simulink subsystem "joystick"  (R2026a)
settings: Solver=VariableStepAuto
undefined symbols (not defined in the file): DiscIntNeverNeededParam, FF_maneuvers, I, P, RSFF_maneuvers, S, T
libraries: slpidlib x2, simulink x1
settings Model: Creator=rubystanton  LastModifiedBy=kjhaydon

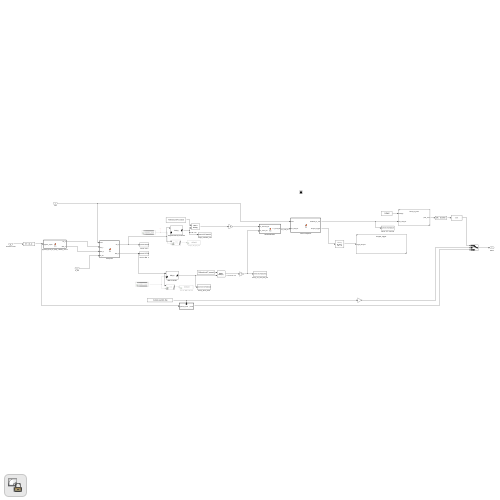
[thumbnail: Simulink's stored preview of the top-level diagram]
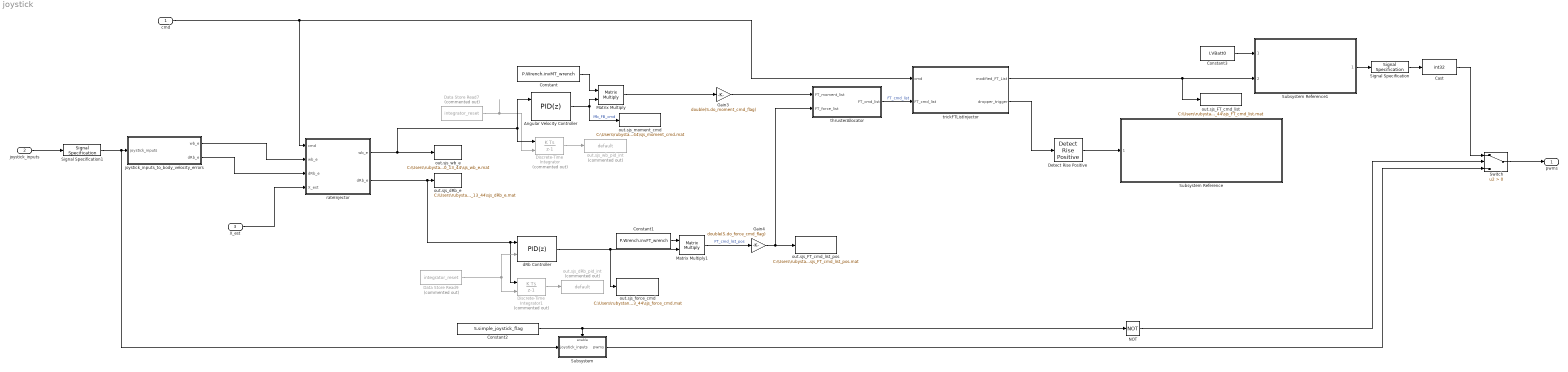
== system joystick ==
  cmd : Inport
  joystick_inputs : Inport  Port=2
  X_est : Inport  Port=3
  Angular Velocity Controller : slpidlib/PID Controller  Controller=PID  Form=Parallel  TimeDomain=Discrete-time  UseExternalTs=off  SampleTime=-1  IntegratorMethod=Forward Euler  FilterMethod=Forward Euler  ControllerParametersSource=internal  P=T.wb_PID.Kp  I=T.wb_PID.Ki  UseKiTs=off  D=T.wb_PID.Kd  UseExternalDerivativeSource=off  N=T.wb_PID.N  UseFilter=on  TunerSelectOption=Transfer Function Based (PID Tuner App)  InitialConditionSource=internal  InitialConditionForIntegrator=0  InitialConditionForFilter=0  DifferentiatorICPrevScaledInput=0  ExternalReset=rising  TrackingMode=off  Kt=1  LimitOutput=on  SatLimitsSource=internal  UpperSaturationLimit=T.wb_PID.output_sat  LowerSaturationLimit=-T.wb_PID.output_sat  LinearizeAsGain=on  AntiWindupMode=clamping  Kb=1  LimitIntegrator=on  UpperIntegratorSaturationLimit=T.wb_PID.int_sat  LowerIntegratorSaturationLimit=-T.wb_PID.int_sat  POutMin=[]  POutMax=[]  IOutMin=[]  IOutMax=[]  DOutMin=[]  DOutMax=[]  NOutMin=[]  NOutMax=[]  SumOutMin=[]  SumOutMax=[]  SaturationOutMin=[]  SaturationOutMax=[]  PParamMin=[]  PParamMax=[]  IParamMin=[]  IParamMax=[]  DParamMin=[]  DParamMax=[]  NParamMin=[]  NParamMax=[]  KbParamMin=[]  KbParamMax=[]  KtParamMin=[]  KtParamMax=[]  KbOutMin=[]  KbOutMax=[]  KtOutMin=[]  KtOutMax=[]  IntegratorOutMin=[]  IntegratorOutMax=[]  FilterOutMin=[]  FilterOutMax=[]  SumI1OutMin=[]  SumI1OutMax=[]  SumI2OutMin=[]  SumI2OutMax=[]  SumI3OutMin=[]  SumI3OutMax=[]  SumI4OutMin=[]  SumI4OutMax=[]  SumDOutMin=[]  SumDOutMax=[]  DifferentiatorOutMin=[]  DifferentiatorOutMax=[]  FilterDiffOutCoefMin=[]  FilterDiffOutCoefMax=[]  ReciprocalOutMin=[]  ReciprocalOutMax=[]  SumDenOutMin=[]  SumDenOutMax=[]  SumNumOutMin=[]  SumNumOutMax=[]  DivideOutMin=[]  DivideOutMax=[]  UdiffTsProdOutMin=[]  UdiffTsProdOutMax=[]  NTsProdOutMin=[]  NTsProdOutMax=[]  UintegralTsProdOutMin=[]  UintegralTsProdOutMax=[]  UngainTsProdOutMin=[]  UngainTsProdOutMax=[]  ClampingZeroOutDataTypeStr=Inherit: Inherit via back propagation  ClampingZeroOutMin=[]  ClampingZeroOutMax=[]  FilterDenConstantOutDataTypeStr=Inherit: Inherit via back propagation  FilterDenConstantOutMin=[]  FilterDenConstantOutMax=[]  PCopyOutDataTypeStr=Inherit: Inherit via back propagation  PCopyOutMin=[]  PCopyOutMax=[]  NCopyOutDataTypeStr=Inherit: Inherit via back propagation  NCopyOutMin=[]  NCopyOutMax=[]  IntegratorContinuousStateAttributes=''  IntegratorStateMustResolveToSignalObject=off  IntegratorRTWStateStorageClass=Auto  FilterContinuousStateAttributes=''  FilterStateMustResolveToSignalObject=off  FilterRTWStateStorageClass=Auto  ParallelPVariant=InternalParameters  IdealPVariant=Disabled  IVariant=InternalParameters  DVariant=InternalParameters  IntegratorVariant=Discrete  SatVariant=Enabled  AWVariant=DiscClampingParallel  PCopyVariant=Disabled  TRVariant=Disabled  FdbkBlocksVariant=Forward  IdealPFdbkVariant=Disabled  SatFdbkVariant=Disabled  DerivativeFilterVariant=ForwardEulerFilter  NVariant=InternalParameters  NCopyVariant=Disabled  FilterICVariant=InternalICsFilter  IntegratorICVariant=InternalICs  ExternalResetVariant=ExternalReset  TRSumVariant=Passthrough  SumFdbkVariant=Disabled  SumVariant=Sum_PID  TsampFilterVariant=InternalTs  TsampNgainVariant=Passthrough  TsampIntegralVariant=Disabled_SignalSpec  ExternalSaturationOutDataTypeStr=Inherit: Same as second input  DerivativeSourceVariant=ErrorSignal  PreIntVariant=InternalPreInt
  Cast : DataTypeConversion  OutDataTypeStr=int32  SaturateOnIntegerOverflow=off  RndMeth=Floor
  Constant : Constant  Value=P.Wrench.invMT_wrench
  Constant1 : Constant  Value=P.Wrench.invFT_wrench
  Constant2 : Constant  Value=S.simple_joystick_flag
  Constant3 : Constant  Value=I.VBatt0
  Data Store Read7 : DataStoreRead  Commented=on  DataStoreName=integrator_reset  IndexOptions=Index vector (dialog)  Indices=1  OutputSizes=1
  Data Store Read9 : DataStoreRead  Commented=on  DataStoreName=integrator_reset  IndexOptions=Index vector (dialog)  Indices=1  OutputSizes=1
  Detect Rise Positive : simulink/Logic and Bit Operations/Detect Rise Positive  vinit=0  OutDataTypeStr=boolean
  Discrete-Time Integrator : DiscreteIntegrator  Commented=on  gainval=T.wb_PID.Ki  ExternalReset=rising  InitialCondition=[0;0;0]  SampleTime=S.dt_control  LimitOutput=on  UpperSaturationLimit=T.wb_PID.int_sat  LowerSaturationLimit=-T.wb_PID.int_sat  ICPrevOutput=DiscIntNeverNeededParam  ICPrevScaledInput=DiscIntNeverNeededParam
  Discrete-Time Integrator1 : DiscreteIntegrator  Commented=on  gainval=T.dRb_PID.Ki  ExternalReset=rising  InitialCondition=[0;0;0]  SampleTime=S.dt_control  LimitOutput=on  UpperSaturationLimit=T.dRb_PID.int_sat  LowerSaturationLimit=-T.dRb_PID.int_sat  ICPrevOutput=DiscIntNeverNeededParam  ICPrevScaledInput=DiscIntNeverNeededParam
  Gain3 : Gain  Gain=double(S.do_moment_cmd_flag)
  Gain4 : Gain  Gain=double(S.do_force_cmd_flag)
  Matrix Multiply : Product  Multiplication=Matrix(*)
  Matrix Multiply1 : Product  Multiplication=Matrix(*)
  NOT : Logic  Operator=NOT  IconShape=distinctive  AllPortsSameDT=off  OutDataTypeStr=boolean
  Signal Specification : SignalSpecification  OutDataTypeStr=double
  Signal Specification1 : SignalSpecification  Dimensions=[6,1]
  Subsystem : Subsystem
  Subsystem Reference : Subsystem  ReferencedSubsystem=dropper_trigger
  Subsystem Reference1 : Subsystem  ReferencedSubsystem=force_to_pwm
  Switch : Switch  Criteria=u2 > Threshold  SaturateOnIntegerOverflow=off  InputSameDT=off
  dRb Controller : slpidlib/PID Controller  Controller=PID  Form=Parallel  TimeDomain=Discrete-time  UseExternalTs=off  SampleTime=-1  IntegratorMethod=Forward Euler  FilterMethod=Forward Euler  ControllerParametersSource=internal  P=T.dRb_PID.Kp  I=T.dRb_PID.Ki  UseKiTs=off  D=T.dRb_PID.Kd  UseExternalDerivativeSource=off  N=T.dRb_PID.N  UseFilter=on  TunerSelectOption=Transfer Function Based (PID Tuner App)  InitialConditionSource=internal  InitialConditionForIntegrator=0  InitialConditionForFilter=0  DifferentiatorICPrevScaledInput=0  ExternalReset=rising  TrackingMode=off  Kt=1  LimitOutput=on  SatLimitsSource=internal  UpperSaturationLimit=T.dRb_PID.output_sat  LowerSaturationLimit=-T.dRb_PID.output_sat  LinearizeAsGain=on  AntiWindupMode=clamping  Kb=1  LimitIntegrator=on  UpperIntegratorSaturationLimit=T.dRb_PID.int_sat  LowerIntegratorSaturationLimit=-T.dRb_PID.int_sat  POutMin=[]  POutMax=[]  IOutMin=[]  IOutMax=[]  DOutMin=[]  DOutMax=[]  NOutMin=[]  NOutMax=[]  SumOutMin=[]  SumOutMax=[]  SaturationOutMin=[]  SaturationOutMax=[]  PParamMin=[]  PParamMax=[]  IParamMin=[]  IParamMax=[]  DParamMin=[]  DParamMax=[]  NParamMin=[]  NParamMax=[]  KbParamMin=[]  KbParamMax=[]  KtParamMin=[]  KtParamMax=[]  KbOutMin=[]  KbOutMax=[]  KtOutMin=[]  KtOutMax=[]  IntegratorOutMin=[]  IntegratorOutMax=[]  FilterOutMin=[]  FilterOutMax=[]  SumI1OutMin=[]  SumI1OutMax=[]  SumI2OutMin=[]  SumI2OutMax=[]  SumI3OutMin=[]  SumI3OutMax=[]  SumI4OutMin=[]  SumI4OutMax=[]  SumDOutMin=[]  SumDOutMax=[]  DifferentiatorOutMin=[]  DifferentiatorOutMax=[]  FilterDiffOutCoefMin=[]  FilterDiffOutCoefMax=[]  ReciprocalOutMin=[]  ReciprocalOutMax=[]  SumDenOutMin=[]  SumDenOutMax=[]  SumNumOutMin=[]  SumNumOutMax=[]  DivideOutMin=[]  DivideOutMax=[]  UdiffTsProdOutMin=[]  UdiffTsProdOutMax=[]  NTsProdOutMin=[]  NTsProdOutMax=[]  UintegralTsProdOutMin=[]  UintegralTsProdOutMax=[]  UngainTsProdOutMin=[]  UngainTsProdOutMax=[]  ClampingZeroOutDataTypeStr=Inherit: Inherit via back propagation  ClampingZeroOutMin=[]  ClampingZeroOutMax=[]  FilterDenConstantOutDataTypeStr=Inherit: Inherit via back propagation  FilterDenConstantOutMin=[]  FilterDenConstantOutMax=[]  PCopyOutDataTypeStr=Inherit: Inherit via back propagation  PCopyOutMin=[]  PCopyOutMax=[]  NCopyOutDataTypeStr=Inherit: Inherit via back propagation  NCopyOutMin=[]  NCopyOutMax=[]  IntegratorContinuousStateAttributes=''  IntegratorStateMustResolveToSignalObject=off  IntegratorRTWStateStorageClass=Auto  FilterContinuousStateAttributes=''  FilterStateMustResolveToSignalObject=off  FilterRTWStateStorageClass=Auto  ParallelPVariant=InternalParameters  IdealPVariant=Disabled  IVariant=InternalParameters  DVariant=InternalParameters  IntegratorVariant=Discrete  SatVariant=Enabled  AWVariant=DiscClampingParallel  PCopyVariant=Disabled  TRVariant=Disabled  FdbkBlocksVariant=Forward  IdealPFdbkVariant=Disabled  SatFdbkVariant=Disabled  DerivativeFilterVariant=ForwardEulerFilter  NVariant=InternalParameters  NCopyVariant=Disabled  FilterICVariant=InternalICsFilter  IntegratorICVariant=InternalICs  ExternalResetVariant=ExternalReset  TRSumVariant=Passthrough  SumFdbkVariant=Disabled  SumVariant=Sum_PID  TsampFilterVariant=InternalTs  TsampNgainVariant=Passthrough  TsampIntegralVariant=Disabled_SignalSpec  ExternalSaturationOutDataTypeStr=Inherit: Same as second input  DerivativeSourceVariant=ErrorSignal  PreIntVariant=InternalPreInt
  joystick_inputs_to_body_velocity_errors : MATLAB Function  TreatAsAtomicUnit=on
  out.sjs_FT_cmd_list : ToFile  Filename=C:\Users\rubystanton\Documents\GitHub\controls-2027\data\2026_10_27_20_13_44\sjs_FT_cmd_list.mat  MatrixName=sjs_FT_cmd_list  SaveFormat=Timeseries  SampleTime=S.dt_data
  out.sjs_FT_cmd_list_pos : ToFile  Filename=C:\Users\rubystanton\Documents\GitHub\controls-2027\data\2026_10_27_20_13_44\sjs_FT_cmd_list_pos.mat  MatrixName=sjs_FT_cmd_list_pos  SaveFormat=Timeseries
  out.sjs_dRb_e : ToFile  Filename=C:\Users\rubystanton\Documents\GitHub\controls-2027\data\2026_10_27_20_13_44\sjs_dRb_e.mat  MatrixName=sjs_dRb_e  SaveFormat=Timeseries  SampleTime=S.dt_data
  out.sjs_dRb_pid_int : ToFile  Commented=on  Filename=default  MatrixName=sjs_dRb_pid_int  SaveFormat=Timeseries  SampleTime=S.dt_data
  out.sjs_force_cmd : ToFile  Filename=C:\Users\rubystanton\Documents\GitHub\controls-2027\data\2026_10_27_20_13_44\sjs_force_cmd.mat  MatrixName=sjs_force_cmd  SaveFormat=Timeseries  SampleTime=S.dt_data
  out.sjs_moment_cmd : ToFile  Filename=C:\Users\rubystanton\Documents\GitHub\controls-2027\data\2026_10_27_20_13_44\sjs_moment_cmd.mat  MatrixName=sjs_moment_cmd  SaveFormat=Timeseries  SampleTime=S.dt_data
  out.sjs_wb_e : ToFile  Filename=C:\Users\rubystanton\Documents\GitHub\controls-2027\data\2026_10_27_20_13_44\sjs_wb_e.mat  MatrixName=sjs_wb_e  SaveFormat=Timeseries  SampleTime=S.dt_data
  out.sjs_wb_pid_int : ToFile  Commented=on  Filename=default  MatrixName=sjs_wb_pid_int  SaveFormat=Timeseries  SampleTime=S.dt_data
  rateInjector : MATLAB Function  TreatAsAtomicUnit=on
  thrusterAllocator : MATLAB Function  TreatAsAtomicUnit=on
  trickFTListInjector : MATLAB Function  TreatAsAtomicUnit=on
  pwms : Outport
  wires:
  trickFTListInjector/2(dropper_trigger) -> Detect Rise Positive/1
  Subsystem/1(pwms) -> Switch/3
  NOT/1 -> Switch/2
  Signal Specification/1 -> Cast/1
  Matrix Multiply/1 -> Gain3/1
  Signal Specification1/1 -> Subsystem/1(joystick_inputs), joystick_inputs_to_body_velocity_errors/1(joystick_inputs)
  Detect Rise Positive/1 -> Subsystem Reference/1
  thrusterAllocator/1(FT_cmd_list) -> trickFTListInjector/2(FT_cmd_list)  "FT_cmd_list"
  Subsystem Reference1/1 -> Signal Specification/1
  Discrete-Time Integrator/1 -> out.sjs_wb_pid_int/1
  Discrete-Time Integrator1/1 -> out.sjs_dRb_pid_int/1
  Switch/1 -> pwms/1
  cmd/1 -> rateInjector/1(cmd), trickFTListInjector/1(cmd)
  Data Store Read7/1 -> Discrete-Time Integrator/2
  X_est/1 -> rateInjector/4(X_est)
  Constant/1 -> Matrix Multiply/1
  Constant2/1 -> NOT/1, Subsystem/Enable
  rateInjector/2(dRb_e) -> out.sjs_dRb_e/1, Discrete-Time Integrator1/1, dRb Controller/1
  dRb Controller/1 -> Matrix Multiply1/2, out.sjs_force_cmd/1
  Angular Velocity Controller/1 -> Matrix Multiply/2, out.sjs_moment_cmd/1  "Mb_FB_cmd"
  Constant3/1 -> Subsystem Reference1/1
  Data Store Read9/1 -> dRb Controller/2, Discrete-Time Integrator1/2
  joystick_inputs_to_body_velocity_errors/1(wb_e) -> rateInjector/2("wb_e ")
  joystick_inputs/1 -> Signal Specification1/1
  Constant1/1 -> Matrix Multiply1/1
  Gain3/1 -> thrusterAllocator/1(FT_moment_list)
  rateInjector/1(wb_e) -> out.sjs_wb_e/1, Discrete-Time Integrator/1, Angular Velocity Controller/1
  joystick_inputs_to_body_velocity_errors/2(dRb_e) -> rateInjector/3("dRb_e ")
  Cast/1 -> Switch/1
  Matrix Multiply1/1 -> Gain4/1  "FT_cmd_list_pos"
  Gain4/1 -> out.sjs_FT_cmd_list_pos/1, thrusterAllocator/2(FT_force_list)
  trickFTListInjector/1(modified_FT_List) -> out.sjs_FT_cmd_list/1, Subsystem Reference1/2

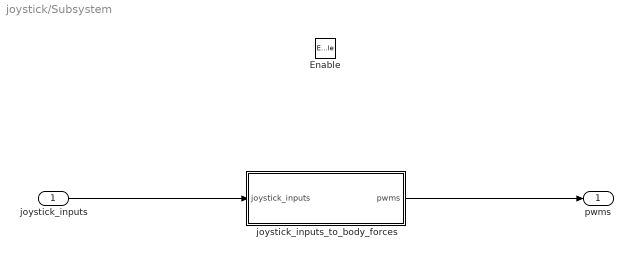
== system joystick/Subsystem ==
  joystick_inputs : Inport
  Enable : EnablePort
  joystick_inputs_to_body_forces : MATLAB Function  TreatAsAtomicUnit=on
  pwms : Outport
  wires:
  joystick_inputs_to_body_forces/1(pwms) -> pwms/1
  joystick_inputs/1 -> joystick_inputs_to_body_forces/1(joystick_inputs)

== matlab function joystick/Subsystem/joystick_inputs_to_body_forces ==
  data: pwms output; joystick_inputs input
%{
Function ported from SimulinkPlant Kory-Work-Branch Mission_Manager_HIL.slx.

Written by Alex Zamora.
%}

function pwms = fcn(joystick_inputs)

%Create the mapping here for PWM values.
%Recall that PWM 1-8 correspond to thruster postions which follow,

%pwm of each thruster on the robot
%In left to right:
%f = front / r = rear
%l = left  / r = right
%t = top   / b = bottom
%PWM(1)=pwm_flt
%PWM(2)=pwm_frt
%PWM(3)=pwm_rlt
%PWM(4)=pwm_rrt
%PWM(5)=pwm_flb
%PWM(6)=pwm_frb
%PWM(7)=pwm_rlb
%PWM(8)=pwm_rrb
  
x_joy = joystick_inputs(1);
y_joy = joystick_inputs(2);
rise = joystick_inputs(3);
sink = joystick_inputs(4);
yaw = joystick_inputs(5);
pitch = joystick_inputs(6);


scale = 300;
stop_set = 1500;
max_pwm = 1500+scale;
min_pwm = 1500-scale;

%x_body and y_body mapping
x = y_joy;
y = x_joy;

pwms_vert = stop_set*ones(1,4); %Thrusters 0,1,2,3
pwms_horiz = stop_set*ones(1,4); %Thrusters 4,5,6,7
inversion_mask = [1, -1, 1, -1];

% Rise/Sink
for i = 1:4
    pwms_vert(i) = pwms_vert(i) + (scale*rise - scale*sink) * inversion_mask(i);
end

%Pitch
pwms_vert(1) = pwms_vert(1) - (scale*pitch*inversion_mask(1));
pwms_vert(2) = pwms_vert(2) - (scale*pitch*inversion_mask(2));
pwms_vert(3) = pwms_vert(3) + (scale*pitch*inversion_mask(3));
pwms_vert(4) = pwms_vert(4) + (scale*pitch*inversion_mask(4));

% Forwards:
pwms_horiz(1) = pwms_horiz(1) + scale*x;
pwms_horiz(2) = pwms_horiz(2) - scale*x;
pwms_horiz(3) = pwms_horiz(3) + scale*x;
pwms_horiz(4) = pwms_horiz(4) - scale*x;

% Strafe:
pwms_horiz(1) = pwms_horiz(1) + y*scale;
pwms_horiz(2) = pwms_horiz(2) + y*scale;
pwms_horiz(3) = pwms_horiz(3) - y*scale;
pwms_horiz(4) = pwms_horiz(4) - y*scale;

% Yaw:
pwms_horiz(1) = pwms_horiz(1) + yaw*scale;
pwms_horiz(2) = pwms_horiz(2) + yaw*scale;
pwms_horiz(3) = pwms_horiz(3) + yaw*scale;
pwms_horiz(4) = pwms_horiz(4) + yaw*scale;


for i = 1:4
    if(pwms_horiz(i) > max_pwm)
        pwms_horiz(i) = max_pwm;
    end
    if(pwms_horiz(i) < min_pwm)
        pwms_horiz(i) = min_pwm;
    end
    if(pwms_vert(i) > max_pwm)
        pwms_vert(i) = max_pwm;
    end
    if(pwms_vert(i) < min_pwm)
        pwms_horiz(i) = min_pwm;
    end

end

pwms = int32([pwms_vert,pwms_horiz])';

== matlab function joystick/joystick_inputs_to_body_velocity_errors ==
  data: wb_e output; joystick_inputs input; T parameter; dRb_e output
function [wb_e,dRb_e]= fcn(joystick_inputs,T)

%Creates velocity errors based on joystick inputs.
x_joy = joystick_inputs(1);
y_joy = joystick_inputs(2);
rise = joystick_inputs(3);
sink = joystick_inputs(4);
yaw = joystick_inputs(5);
pitch = joystick_inputs(6);

%sensitivities
r_sensitivity = T.js_wb_e;
t_sensitivity = T.js_dRb_e;

%x_body and y_body mapping
x = y_joy;
y = x_joy;

wb_e = [0 0 0]';
dRb_e = [0 0 0]';

%translation
dRb_e(1)=t_sensitivity(2-logical(1+sign(x)),1)*x;
dRb_e(2)=t_sensitivity(2-logical(1+sign(y)),2)*y;
z = sink-rise;
dRb_e(3)=t_sensitivity(2-logical(1+sign(z)),3)*z;

%rotation
wb_e(2) = r_sensitivity(2-logical(1+sign(pitch)),2)*pitch;
wb_e(3) = r_sensitivity(2-logical(1+sign(yaw)),3)*yaw;

== matlab function joystick/rateInjector ==
  data: cmd input Bus: cmd_bus; wb_e input; wb_e output; dRb_e input; dRb_e output; RSFF_maneuvers parameter Bus: RSFF_maneuver_bus; X_est input Bus: X_bus; S parameter
function [wb_e, dRb_e] = fcn(cmd, wb_e, dRb_e, RSFF_maneuvers, X_est, S)

overwrite_rate_error_flag = S.overwrite_rate_error_flag;
wb_error_inject = S.wb_error_inject;
dRb_error_inject = S.dRb_error_inject;
[wb_e, dRb_e] = rateInjector(cmd, wb_e, dRb_e, X_est, RSFF_maneuvers, overwrite_rate_error_flag, wb_error_inject, dRb_error_inject);

== matlab function joystick/thrusterAllocator ==
  data: FT_moment_list input; FT_cmd_list output; FT_force_list input; P parameter
function FT_cmd_list = fcn(FT_moment_list, FT_force_list, P)

max_thruster_force = P.Constants.max_thruster_force;

FT_cmd_list = thrusterAllocator(FT_moment_list, FT_force_list, max_thruster_force);

== matlab function joystick/trickFTListInjector ==
  data: cmd input; modified_FT_List output size=[8,1]; FT_cmd_list input; FF_maneuvers parameter Bus: FF_maneuvers_bus; S parameter; dropper_trigger output
function [modified_FT_List, dropper_trigger] = fcn(cmd, FT_cmd_list, FF_maneuvers,S)

overwrite_FT_list_flag = S.overwrite_FT_list_flag;
FT_list_inject = S.FT_list_inject;

[modified_FT_List, dropper_trigger] = trickFTListInjector(cmd, FT_cmd_list, FF_maneuvers, overwrite_FT_list_flag, FT_list_inject);
